simulink model "normal"  (R2020a)
settings: Solver=ode45  StartTime=0.0  StopTime=0.4  FixedStep=1e-6  MaxStep=0.04  RelTol=1e-3  EnableMultiTasking=on
PreLoadFcn:
  | power_13NodeTestFeeder_init;
values from neighbouring files (symbols this model uses):
  C_601 = [1.03835973183e-08  -3.28956213337e-09  -2.07596127216e-09; -3.28956213337e-09  9.8230300863e-09  -1.22250137004e-09; -2.07596127216e-09  -1.22250137004e-09  9.29377945947e-09]    [Finalmat.mat]    (also in bus1.mat; bus10.mat; bus11.mat; bus12.mat)
  C_602 = [9.39333329896e-09  -1.78290377777e-09  -2.78635373607e-09; -1.78290377777e-09  8.5370713848e-09  -1.08586207709e-09; -2.78635373607e-09  -1.08586207709e-09  8.94105559107e-09]    [Finalmat.mat]    (also in bus1.mat; bus10.mat; bus11.mat; bus12.mat)
  C_603 = [0  0  0; 0  7.76272711671e-09  -1.48325331387e-09; 0  -1.48325331387e-09  7.69036927641e-09]    [Finalmat.mat]    (also in bus1.mat; bus10.mat; bus11.mat; bus12.mat)
  C_604 = [7.69036927641e-09  0  -1.48325331387e-09; 0  0  0; -1.48325331387e-09  0  7.76272711671e-09]    [Finalmat.mat]    (also in bus1.mat; bus10.mat; bus11.mat; bus12.mat)
  C_605 = [0  0  0; 0  0  0; 0  0  7.44890176838e-09]    [Finalmat.mat]    (also in bus1.mat; bus10.mat; bus11.mat; bus12.mat)
  C_606 = [1.59697709306e-07  -1.64824237567e-15  -1.64824237567e-15; -1.64824237567e-15  1.59697709306e-07  -1.64824237567e-15; -1.64824237567e-15  -1.64824237567e-15  1.59697709306e-07]    [Finalmat.mat]    (also in bus1.mat; bus10.mat; bus11.mat; bus12.mat)
  C_607 = [1.46679066902e-07  0  0; 0  0  0; 0  0  0]    [Finalmat.mat]    (also in bus1.mat; bus10.mat; bus11.mat; bus12.mat)
  ft2km = 0.0003048    [Finalmat.mat]    (also in bus1.mat; bus10.mat; bus11.mat; bus12.mat)
  L_601 = [0.0016777459142  0.000826923199875  0.000698195470335; 0.000826923199875  0.00172702836123  0.000634408490396; 0.000698195470335  0.000634408490396  0.00170560121035]    [Finalmat.mat]    (also in bus1.mat; bus10.mat; bus11.mat; bus12.mat)
  L_602 = [0.00194723354262  0.000698195470335  0.000826923199875; 0.000698195470335  0.00197508883877  0.000634408490396; 0.000826923199875  0.000634408490396  0.00199635116541]    [Finalmat.mat]    (also in bus1.mat; bus10.mat; bus11.mat; bus12.mat)
  L_603 = [0  0  0; 0  0.00222034730427  0.000756708074671; 0  0.000756708074671  0.00223650007955]    [Finalmat.mat]    (also in bus1.mat; bus10.mat; bus11.mat; bus12.mat)
  L_604 = [0.00223650007955  0  0.000756708074671; 0  0  0; 0.000756708074671  0  0.00222034730427]    [Finalmat.mat]    (also in bus1.mat; bus10.mat; bus11.mat; bus12.mat)
  L_605 = [0  0  0; 0  0  0; 0  0  0.00222100660122]    [Finalmat.mat]    (also in bus1.mat; bus10.mat; bus11.mat; bus12.mat)
  L_606 = [0.000735610572263  5.40623499221e-05  2.35698659721e-05; 5.40623499221e-05  0.000666054744009  5.40623499221e-05; 2.35698659721e-05  5.40623499221e-05  0.000735610572263]    [Finalmat.mat]    (also in bus1.mat; bus10.mat; bus11.mat; bus12.mat)
  L_607 = [0.000844559393295  0  0; 0  0  0; 0  0  0]    [Finalmat.mat]    (also in bus1.mat; bus10.mat; bus11.mat; bus12.mat)
  R_601 = [0.215305653249  0.0969341469174  0.0981768923907; 0.0969341469174  0.209713298619  0.0953807150757; 0.0981768923907  0.0953807150757  0.212136652292]    [Finalmat.mat]    (also in bus1.mat; bus10.mat; bus11.mat; bus12.mat)
  R_602 = [0.467645121603  0.0981768923907  0.0969341469174; 0.0981768923907  0.464476120646  0.0953807150757; 0.0969341469174  0.0953807150757  0.462052766973]    [Finalmat.mat]    (also in bus1.mat; bus10.mat; bus11.mat; bus12.mat)
  R_603 = [0  0  0; 0  0.826052916102  0.128375607392; 0  0.128375607392  0.822573228777]    [Finalmat.mat]    (also in bus1.mat; bus10.mat; bus11.mat; bus12.mat)
  R_604 = [0.822573228777  0  0.128375607392; 0  0  0; 0.128375607392  0  0.826052916102]    [Finalmat.mat]    (also in bus1.mat; bus10.mat; bus11.mat; bus12.mat)
  R_605 = [0  0  0; 0  0  0; 0  0  0.825928641555]    [Finalmat.mat]    (also in bus1.mat; bus10.mat; bus11.mat; bus12.mat)
  R_606 = [0.495979718394  0.198342177539  0.177029092672; 0.198342177539  0.49032522649  0.198342177539; 0.177029092672  0.198342177539  0.495979718394]    [Finalmat.mat]    (also in bus1.mat; bus10.mat; bus11.mat; bus12.mat)
  R_607 = [0.834192898952  0  0; 0  0  0; 0  0  0]    [Finalmat.mat]    (also in bus1.mat; bus10.mat; bus11.mat; bus12.mat)
libraries: neural x322, powerlib x54, powerlib_meascontrol x6, simulink x1
(part 4 of 8)

== system normal/Subsystem1/Function Fitting Neural Network/Layer 2/Delays 1 ==
  "p{2}" : Inport  PortDimensions=100
      mask Display: e = 0.06;c1 = [120 230 180]/255;c2 = ([120 230 180]+0)/(256+128);c3 = ([120 230 180]+128)/(256+128);patch([0 1 1 0],[0 0 1 1],c1);patch([0 1 1 1-e 1-e 0+e],[0 0 1 1-e 0+e 0+e],c2);patch([0 0 1 1-e 0+e 0+e],[0 1 1 1-e 1-e 0+e],c3);plot([0 1 1 0 0],[0 0 1 1 0]);
  mux : Mux  Inputs=1
      mask Display: e = 0.06;c1 = [120 150 230]/255;c2 = ([120 150 230]+0)/383;c3 = ([120 150 230]+128)/383;patch([0 1 1 0],[0 0 1 1],c1);patch([0 1 1 1-e 1-e 0+e],[0 0 1 1-e 0+e 0+e],c2);patch([0 0 1 1-e 0+e 0+e],[0 1 1 1-e 1-e 0+e],c3);plot([0 1 1 0 0],[0 0 1 1 0]);disp('Mux')
  "pd{2,1}" : Outport
      mask Display: e = 0.06;c1 = [120 230 180]/255;c2 = ([120 230 180]+0)/(256+128);c3 = ([120 230 180]+128)/(256+128);patch([0 1 1 0],[0 0 1 1],c1);patch([0 1 1 1-e 1-e 0+e],[0 0 1 1-e 0+e 0+e],c2);patch([0 0 1 1-e 0+e 0+e],[0 1 1 1-e 1-e 0+e],c3);plot([0 1 1 0 0],[0 0 1 1 0]);
  wires:
  "p{2}"/1 -> mux/1
  mux/1 -> "pd{2,1}"/1

== system normal/Subsystem1/Function Fitting Neural Network/Layer 2/LW{2,1} ==
  "ad{2,1}" : Inport  PortDimensions=100
      mask Display: e = 0.06;c1 = [120 230 180]/255;c2 = ([120 230 180]+0)/(256+128);c3 = ([120 230 180]+128)/(256+128);patch([0 1 1 0],[0 0 1 1],c1);patch([0 1 1 1-e 1-e 0+e],[0 0 1 1-e 0+e 0+e],c2);patch([0 0 1 1-e 0+e 0+e],[0 1 1 1-e 1-e 0+e],c3);plot([0 1 1 0 0],[0 0 1 1 0]);
  "IW{2,1}(1,:)'" : Constant  Value=[1.8793908287279783575485225810552947223186492919921875;-0.9048667518245905316831567688495852053165435791015625;-0.92458538808867185565532054170034825801849365234375;-2.02532521067546245063795140595175325870513916015625;5.33525657670273556476558951544575393199920654296875;3.210800612231773154547909143730066716670989990234375;-0.09324484938112427567791229421345633454620838165283203125;0.03540388689183378290170622904042829759418964385986328125;0.1885587765727710640728531643617316149175167083740234375;-4.22107099118371120738402169081382453441619873046875;-0.264501726010362647745211006622412241995334625244140625;-0.34225779722053040199369888796354644000530242919921875;-0.373202417779953388166092054234468378126621246337890625;8.2600182662194896465734927915036678314208984375;-3.2632258813898840088540964643470942974090576171875;-0.62922711116860108315762545316829346120357513427734375;-0.38755461469218255299296060911729000508785247802734375;0.65203344442902988475907477550208568572998046875;-2.26821878466440285393446174566633999347686767578125;0.543177487170682926631570808240212500095367431640625;-2.789913530456374690658094550599344074726104736328125;0.1798698221775162642277479108088300563395023345947265625;0.399305983587987689542586622337694279849529266357421875;1.2306887105144139749057785593322478234767913818359375;1.456708317179773448657442713738419115543365478515625;1.035561461053104093110732719651423394680023193359375;0.27441751827051164003279382086475379765033721923828125;-0.204970973074732831786803899376536719501018524169921875;-0.253112822104407164669481744567747227847576141357421875;0.1510518587617716013138391417669481597840785980224609375;-0.31745069317599250435790736446506343781948089599609375;-0.676791919103845618366221970063634216785430908203125;-2.978627056642336068392751258215866982936859130859375;9.0535751730324189878729157499037683010101318359375;-8.190932561555936075592398992739617824554443359375;0.49841770298888565804418249172158539295196533203125;-0.50061513193962159373739950751769356429576873779296875;1.53295551447780287190880699199624359607696533203125;12.583976878439415258981171064078807830810546875;-0.09178682720573481945702809525755583308637142181396484375;8.636594135212391165623557753860950469970703125;3.910230596444252970655952594825066626071929931640625;-2.50969331155198016602980715106241405010223388671875;-0.32572264372845494140307209818274714052677154541015625;2.658418596062821048775504095829091966152191162109375;4.26885657500254556140362183214165270328521728515625;1.4483077928253802468816502369008958339691162109375;-1.0548868080331390562065507765510119497776031494140625;-1.75700921521880726317021981230936944484710693359375;-4.8518766072740096007009924505837261676788330078125;-0.043810031439321835133871019252183032222092151641845703125;0.418247245768505415686178139367257244884967803955078125;-1.54235777001860352442008661455474793910980224609375;0.2440732320832143809052894312117132358253002166748046875;-2.981478415506142010116263918462209403514862060546875;-0.1983812993079519804151544803971773944795131683349609375;-0.488626450603534212557832461243378929793834686279296875;-4.16709607961305028567267072503454983234405517578125;2.59533520027240083294373107491992413997650146484375;4.20601887646172389878529429552145302295684814453125;3.531120270555935025669214155641384422779083251953125;-0.51904717173316872180777181711164303123950958251953125;1.751606913577048896257792875985614955425262451171875;2.297924274586310655621446130680851638317108154296875;0.10235191318978331675992876625969074666500091552734375;0.68318748611821000782384771810029633343219757080078125;1.0577758447114204987116181655437685549259185791015625;3.15370331022145489185959377209655940532684326171875;1.325141327935329460530056167044676840305328369140625;4.03421651104892742267793437349610030651092529296875;-9.5505906993198106391673718462698161602020263671875;-0.21252767811685158161338904392323456704616546630859375 ...(+1553 chars)]
      mask Display: e = 0.06;c1 = [120 150 230]/255;c2 = ([120 150 230]+0)/383;c3 = ([120 150 230]+128)/383;patch([0 1 1 0],[0 0 1 1],c1);patch([0 1 1 1-e 1-e 0+e],[0 0 1 1-e 0+e 0+e],c2);patch([0 0 1 1-e 0+e 0+e],[0 1 1 1-e 1-e 0+e],c3);plot([0 1 1 0 0],[0 0 1 1 0]);disp('weights');
  Mux : Mux  Inputs=1
      mask Display: e = 0.06;c1 = [120 150 230]/255;c2 = ([120 150 230]+0)/383;c3 = ([120 150 230]+128)/383;patch([0 1 1 0],[0 0 1 1],c1);patch([0 1 1 1-e 1-e 0+e],[0 0 1 1-e 0+e 0+e],c2);patch([0 0 1 1-e 0+e 0+e],[0 1 1 1-e 1-e 0+e],c3);plot([0 1 1 0 0],[0 0 1 1 0]);disp('Mux');
  dotprod1 : neural/Weight Functions/dotprod
  "lz{2,1}" : Outport
      mask Display: e = 0.06;c1 = [120 230 180]/255;c2 = ([120 230 180]+0)/(256+128);c3 = ([120 230 180]+128)/(256+128);patch([0 1 1 0],[0 0 1 1],c1);patch([0 1 1 1-e 1-e 0+e],[0 0 1 1-e 0+e 0+e],c2);patch([0 0 1 1-e 0+e 0+e],[0 1 1 1-e 1-e 0+e],c3);plot([0 1 1 0 0],[0 0 1 1 0]);
  wires:
  "IW{2,1}(1,:)'"/1 -> dotprod1/1
  "ad{2,1}"/1 -> dotprod1/2
  dotprod1/1 -> Mux/1
  Mux/1 -> "lz{2,1}"/1

== system normal/Subsystem1/Function Fitting Neural Network1/Layer 1/Delays 1 ==
  "p{1}" : Inport  PortDimensions=9
      mask Display: e = 0.06;c1 = [120 230 180]/255;c2 = ([120 230 180]+0)/(256+128);c3 = ([120 230 180]+128)/(256+128);patch([0 1 1 0],[0 0 1 1],c1);patch([0 1 1 1-e 1-e 0+e],[0 0 1 1-e 0+e 0+e],c2);patch([0 0 1 1-e 0+e 0+e],[0 1 1 1-e 1-e 0+e],c3);plot([0 1 1 0 0],[0 0 1 1 0]);
  mux : Mux  Inputs=1
      mask Display: e = 0.06;c1 = [120 150 230]/255;c2 = ([120 150 230]+0)/383;c3 = ([120 150 230]+128)/383;patch([0 1 1 0],[0 0 1 1],c1);patch([0 1 1 1-e 1-e 0+e],[0 0 1 1-e 0+e 0+e],c2);patch([0 0 1 1-e 0+e 0+e],[0 1 1 1-e 1-e 0+e],c3);plot([0 1 1 0 0],[0 0 1 1 0]);disp('Mux')
  "pd{1,1}" : Outport
      mask Display: e = 0.06;c1 = [120 230 180]/255;c2 = ([120 230 180]+0)/(256+128);c3 = ([120 230 180]+128)/(256+128);patch([0 1 1 0],[0 0 1 1],c1);patch([0 1 1 1-e 1-e 0+e],[0 0 1 1-e 0+e 0+e],c2);patch([0 0 1 1-e 0+e 0+e],[0 1 1 1-e 1-e 0+e],c3);plot([0 1 1 0 0],[0 0 1 1 0]);
  wires:
  "p{1}"/1 -> mux/1
  mux/1 -> "pd{1,1}"/1
